simulink model "I2C_test_simple2"  (Simulink 7.7)
settings: Solver=FixedStepDiscrete  StartTime=0.0  StopTime=10.0  FixedStep=0.001  RelTol=1e-3
undefined symbols (not defined in the file or in its folder): High
libraries: dsPICdrivers x3, dspswit3 x1
settings Model: Creator=ij8977  LastModifiedBy=ij8977
settings OptimizationCC: OptimizeModelRefInitCode=on  LifeSpan=1
settings RTWCC: SystemTargetFile=pic32.tlc  MakeCommand=make_CreateMPLAB  TemplateMakefile=pic32_gcc.tmf  PostCodeGenCommand=dsPIC_Compile()  Description=Embedded Target for Microchip dsPIC (real-time)  ProcessScript=pic32_make_rtw_hook
settings CodeAppCC: IgnoreCustomStorageClasses=off
settings STFCustomTargetCC: FunctionExecutionProfile=off  IncludeMdlTerminateFcn=off  CombineOutputUpdateFcns=on  SuppressErrorStatus=on  ERTCustomFileBanners=on  SupportContinuousTime=off  SupportNonInlinedSFcns=off  SystemTargetFile=pic32.tlc
settings ERTTargetCC: FunctionExecutionProfile=off  MultiwordLength=2048  ParMdlRefBuildCompliant=off  CompOptLevelCompliant=off  IncludeMdlTerminateFcn=off  SuppressErrorStatus=on  ERTFirstTimeCompliant=off  ModelStepFunctionPrototypeControlCompliant=off  CPPClassGenCompliant=off  InlinedParameterPlacement=NonHierarchical  ERTSrcFileBannerTemplate=dsPIC_code_template.cgt  ERTHdrFileBannerTemplate=dsPIC_code_template.cgt  ERTDataSrcFileTemplate=dsPIC_code_template.cgt  ERTDataHdrFileTemplate=dsPIC_code_template.cgt  ERTCustomFileTemplate=dsPIC_main.tlc  ConvertIfToSwitch=off
settings CustomProperty: DataType=string  Value=C:\Users\ij8977\Desktop\MATLAB~1\bin\win32\gmake

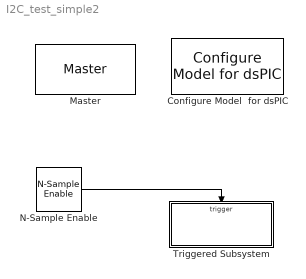
== system I2C_test_simple2 ==
  Configure Model  for dsPIC : dsPICdrivers/Simulink Configuration/Configure Model  for dsPIC
  Master : dsPICdrivers/Master  Tag=dsPIC_MASTER  Priority=1  TimeStepType=Timer1  picType=32MX320F128H  fcy=234375  Quartz_33f=8e6  PLLActive_33f=off  fcyDesired_33f=0  tmr1="[1  233  0.16]"  tmr1Info="Time Step : 0.0009984  ;   Error : 0.16%  PR1=233"  tmr2345="[0  0  0  0]"  tmr2345cfg=[-1 -1 -1 -1]  IOautoConf=on  typePort="[ 0   0   0   0   0   0   0   0   0   0   0   0   0   0   0   0   0   0   0   0   0   0   0   0   0   0   0   0   0   0   0   0   0   0   0   0   0   0   0   0   0   0   0   0   0   0   0   0   0   0   0   0   0   0   0   0   0   0   0   0   0   0   0   0   0   0   0   0   0   0   0   0   0   0   0   0   0   0   0   0   0   0   0   0   0   0   0   0   0   0   0   0   0   0   0   0   0   0  20  20   0   0   0   0   0   0   0   0   0   0   0   0 ]"  TRIS="[ 65535  65535  65535  65535  65535  65535  65535 ]"  ADPCFG=0  MasterBusyPort=None  MasterOverloadPort=None  FOSC=Quartz (XT - HS)  ClockSwitchMonitor=Both disabled  TempProtection_33f=TEMP_ON  FPBOR=<empty>  PWRT=disable  MCLR=<empty>  ICD=ICS_PGD1  JTAGEN=JTAGEN_OFF  PowerSave=off  OverrideFcy=off  NewFcy=1e6  PR2345="[65535  65535  65535  65535]"
  N-Sample Enable : dspswit3/N-Sample Enable  N=5  ActiveLevel=High (1)  reset=off  TriggerType=Rising edge  Ts=.1  DataType=Logical
  Triggered Subsystem : Subsystem  TreatAsAtomicUnit=on
  wires:
  N-Sample Enable/1 -> Triggered Subsystem/Trigger

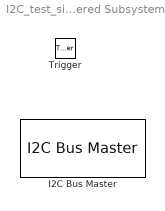
== system I2C_test_simple2/Triggered Subsystem ==
  Trigger : TriggerPort
  I2C Bus Master : dsPICdrivers/BUS I2C/I2C Bus Master  Tag=dsPIC_I2C_Master  NumI2C=1  AltI2C=off  Sequence='S A104 W44 W86 P'  InitializeOnceOnly=When PIC is initialized (only once)  Enable=on  WaitAfterEnable=1  Disable=off  AdressNbrBits=7 bits  I2CBusFreq=100  SlewRate=off  SMBUSThreshold=off  OutputErrorFlag=off  SampleTime=-1  OrderingInOutPopup=None  Info=Fscl = 2315.7082 Hz
